simulink library "Model_DG_Grid_Forming_Converter"  (R2022b)
settings: Solver=VariableStepAuto  StartTime=0.0  StopTime=10.0  RelTol=1e-3
settings Model: Creator=winkens  LastModifiedBy=winkens
settings SolverCC: AlgebraicLoopSolver=TrustRegion
settings DebuggingCC: UnconnectedInputMsg=warning  UnconnectedOutputMsg=warning  UnconnectedLineMsg=warning  SFMachineParentedDataDiag=warning
settings ModelReferenceCC: EnableRefExpFcnMdlSchedulingChecks=on
settings RTWCC: DLArmComputeVersion=19.05

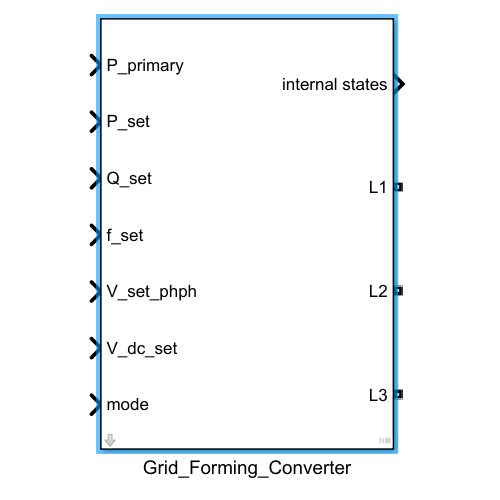
[thumbnail: Simulink's stored preview of the top-level diagram]
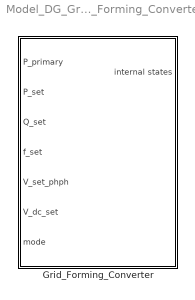
== system Model_DG_Grid_Forming_Converter ==
  Grid_Forming_Converter : Subsystem  mask{S_n=2e6, V_n_phph=690, f_n=50, send_messages=on, T_s_ctrl=1e-4, T_s_PWM_meas=1e-4, T_s_SPS=1e-4, datatype='double', swModeling=Average Model, f_sw=5e3, L_filter_conv_pu=[ 0.001 0.05097 ], C_filter_pu=[ 0.06875 0.04569 ], L_filter_grid_pu=[ 0.01 0.04 ], C_dc_pu=0.75, withTransformer=Grid coupling using transformer, V_n_grid_phph=20e3, RL_Trafo_Conv=[ 0.005 0.02 ], RL_Trafo_Grid=[ 0.005 0.02 ], Rm=500, Lm=500, meas_lowpass=on, meas_f_cutoff_lowpass=2500, meas_f_cutoff_posseq=20, prot_variant=VDE AR, v_dc_max=1.2, v_ac_max=1.4, t_ac_max=0.1, v_ac_maxmax=1.25, t_ac_maxmax=0.1, v_ac_min=0.8, t_ac_min=3, v_ac_minmin=0.45, t_ac_minmin=0.3, f_ac_max=51.5, t_f_ac_max=0.1, f_ac_maxmax=52.5, t_f_ac_maxmax=10, f_ac_min=47.5, t_f_ac_min=0.1, i_ac_max=1.3, outerCtrlStrategy=Droop, OuterCtrl_droop_kP=0.05, OuterCtrl_droop_kQ=0.1, OuterCtrl_droop_TQ=0.2, OuterCtrl_ZDroop_kf=0.05, OuterCtrl_ZDroop_kV=0.1, OuterCtrl_ZDroop_kR=0, OuterCtrl_ZDroop_kX=1, OuterCtrl_ZDroop_TV=0.2, OuterCtrl_VSM_H=0.1, OuterCtrl_VSM_Kd=40, OuterCtrl_VSM_K=20, OuterCtrl_VSM_kQ=0.1, OuterCtrl_VSM_TQ=0.2, OuterCtrl_Dual_Kp=0.01, OuterCtrl_Dual_Kd=1e-4, OuterCtrl_Dual_kQ=0.1, OuterCtrl_Dual_TQ=0.2, OuterCtrl_Lvirt=0, InnerCtrl_K_p_V_cap_controller=0.8, InnerCtrl_K_i_V_cap_controller=0.5, InnerCtrl_K_p_I_conv_controller=3.3, InnerCtrl_K_i_I_conv_controller=16.5, InnerCtrl_v_conv_max=1.3, InnerCtrl_i_conv_max=1, InnerCtrl_Cff_V_cap_ctrl=disabled, InnerCtrl_Cff_I_conv_ctrl=disabled, InnerCtrl_K_ff_I_grid=enabled, InnerCtrl_K_ff_V_cap=enabled, InnerCtrl_i_lim_type=dq coordinate system, InnerCtrl_active_damping=enabled, InnerCtrl_AD_R_virt_pu=0.2}
      mask prompts: S_n "Nominal Apparent Power [VA]"; V_n_phph "Nominal Converter Voltage (rms, phase-to-phase) [V]"; f_n "Nominal Frequency [Hz]"; send_messages "Send tDMSquared info messages"; T_s_ctrl "Controller sample time [s]"; T_s_PWM_meas "PWM and measurements sample time [s]"; T_s_SPS "Simscape SPS sample time [s]"; datatype "Signal data type"; swModeling "Model type:"; f_sw "Switching Frequency [Hz]:"; L_filter_conv_pu "Impedance of Converter-Side-Inductor [ R L ] (p.u.)"; C_filter_pu "Impedance of Filter Capacitor [ R C ] (p.u.)"; L_filter_grid_pu "Impedance of Grid-Side-Inductor* [ R L ] (p.u.)"; C_dc_pu "Capacitance of DC-Side-Capacitor [p.u.]"; V_n_grid_phph "Nominal Grid Voltage (rms, phase-to-phase) [V]"; RL_Trafo_Conv "Converter-Side Impedance [ R L ] (pu):"; RL_Trafo_Grid "Grid-Side Impedance [ R L ] (pu):"; Rm "Magnetization resistance Rm (pu):"; Lm "Magnetization inductance Lm (pu):"; meas_lowpass "Apply low pass filtering to measured signals"; meas_f_cutoff_lowpass "Cutoff-frequency of low pass filter applied to measurement signals [Hz]"; meas_f_cutoff_posseq "Cutoff-frequency of low pass filter for pos. sequence calculation [Hz]"; prot_variant "Protection Variant"; v_dc_max "Maximum DC-link voltage [% nom. value]"; v_ac_max "Maximum AC voltage [% nom. value]"; t_ac_max "Maximum AC voltage timing [s]"; v_ac_maxmax "Upper Maximum AC voltage [% nom. value]"; t_ac_maxmax "Upper Maximum AC voltage timing [s]"; v_ac_min "Upper Minimum AC voltage [% nom. value]"; t_ac_min "Upper Minimum AC voltage timing [s]"; v_ac_minmin "Lower Minimum AC voltage [% nom. value]"; t_ac_minmin "Lower Minimum AC voltage timing [s]"; f_ac_max "Maximum AC frequency[Hz]"; t_f_ac_max "Maximum AC frequency timing [s]"; f_ac_maxmax "Upper Maximum AC frequency [Hz]"; t_f_ac_maxmax "Upper Maximum AC frequency timing [s]"; f_ac_min "Minimum AC frequency [Hz]"; t_f_ac_min "Minimum AC frequency timing [s]"; i_ac_max "Maximum AC current [% nom. value]"; outerCtrlStrategy "Grid-Forming Control Strategy"; OuterCtrl_droop_kP "Droop constant kP (df[pu]/dP[pu])"; OuterCtrl_droop_kQ "Droop constant kQ (dV[pu]/dQ[pu])"; OuterCtrl_droop_TQ "PT1 time constant for QV-loop [s]"; OuterCtrl_ZDroop_kf "Droop constant kf (df/(dP+dQ))"; OuterCtrl_ZDroop_kV "Droop constant kV (dV/(dP+dQ))"; OuterCtrl_ZDroop_kR "R/Z-ratio"; OuterCtrl_ZDroop_kX "X/Z-ratio"; OuterCtrl_ZDroop_TV "PT1 time constant for voltage loop [s]"; OuterCtrl_VSM_H "Virtual inertia [s]"; OuterCtrl_VSM_Kd "Damping constant Kd [pu]"; OuterCtrl_VSM_K "Droop constant (dT/df) [pu]"; OuterCtrl_VSM_kQ "Droop constant kQ (dV/dQ)"; OuterCtrl_VSM_TQ "PT1 time constant QV-loop TQ [s]"; OuterCtrl_Dual_Kp "Proportional gain [pu]"; OuterCtrl_Dual_Kd "Derivative gain [pu]"; OuterCtrl_Dual_kQ "Droop constant kQ (dV/dQ)"; OuterCtrl_Dual_TQ "PT1 time constant QV-loop TQ [s]"; OuterCtrl_Lvirt "Virtual output inductance [pu]"; InnerCtrl_K_p_V_cap_controller "Proportional Gain (PI Voltage Controller)"; InnerCtrl_K_i_V_cap_controller "Integral Gain (PI Voltage Controller)"; InnerCtrl_K_p_I_conv_controller "Proportional Gain (PI Current Controller)"; InnerCtrl_K_i_I_conv_controller "Integral Gain (PI Current Controller)"; InnerCtrl_v_conv_max "Converter voltage maximum value (limit) [p.u.]"; InnerCtrl_i_conv_max "Converter current maximum value (limit) [p.u.]"; InnerCtrl_Cff_V_cap_ctrl "Command-feed-forward (Voltage Controller):"; InnerCtrl_Cff_I_conv_ctrl "Command-feed-forward (Current Controller):"; InnerCtrl_K_ff_I_grid "Current-feed-forward (Voltage Controller):"; InnerCtrl_K_ff_V_cap "Voltage-feed-forward (Current Controller):"; InnerCtrl_i_lim_type "Coordinate system of current setpoint limiter:"; InnerCtrl_active_damping "Active Damping"; InnerCtrl_AD_R_virt_pu "Virtual resistor (in series with converter-side inductance) [p.u.]"
      mask init:
      | % Initialize nominal grid voltage
      | if (withTransformer == 1)
      |     V_n_grid_phph = V_n_phph;
      | end
      mask TypeOptions swModeling: Ideal Switches | Average Model
      mask TypeOptions withTransformer: Direct grid coupling of converter | Grid coupling using transformer
      mask Callback withTransformer:
      | msk = Simulink.Mask.get(gcb);
      | p = msk.Parameters;
      | if strcmp(get_param(gcb, 'withTransformer'), 'Grid coupling using transformer')
      |     %with Transformer
      |     p(16).Visible = 'on';
      |     p(17).Visible = 'on';
      |     p(18).Visible = 'on';
      |     p(19).Visible = 'on';
      |     p(20).Visible = 'on';
      | else
      |     %without Transformer
      |     p(16).Visible = 'off';
      |     p(17).Visible = 'off';
      |     p(18).Visible = 'off';
      |     p(19).Visible = 'off';
      |     p(20).Visible = 'off';
      | end
      mask TypeOptions prot_variant: Hardware protection | tDMSquared warnings only | deactivated | VDE AR
      mask Callback prot_variant:
      | msk = Simulink.Mask.get(gcb);
      | if strcmp(get_param(gcb, 'prot_variant'), 'VDE AR')
      |     msk.getParameter('v_ac_max').Visible ='on';
      |     msk.getParameter('i_ac_max').Visible ='on';
      |     msk.getParameter('t_ac_max').Visible = 'on';
      |     msk.getParameter('v_ac_maxmax').Visible = 'on';
      |     msk.getParameter('t_ac_maxmax').Visible = 'on';
      |     msk.getParameter('v_ac_min').Visible = 'on';
      |     msk.getParameter('t_ac_min').Visible = 'on';
      |     msk.getParameter('v_ac_minmin').Visible = 'on';
      |     msk.getParameter('t_ac_minmin').Visible = 'on';
      |     msk.getParameter('f_ac_max').Visible = 'on';
      |     msk.getParameter('t_f_ac_max').Visible = 'on';
      |     msk.getParameter('f_ac_maxmax').Visible = 'on';
      |     msk.getParameter('t_f_ac_maxmax').Visible = 'on';
      |     msk.getParameter('f_ac_min').Visible = 'on';
      |     msk.getParameter('t_f_ac_min').Visible = 'on';
      | elseif strcmp(get_param(gcb, 'prot_variant'), 'deactivated')
      |     msk.getParameter('v_ac_max').Visible ='off';
      |     msk.getParameter('i_ac_max').Visible ='off';
      |     msk.getParameter('t_ac_max').Visible = 'off';
      |     msk.getParameter('v_ac_maxmax').Visible = 'off';
      |     msk.getParameter('t_ac_maxmax').Visible = 'off';
      |     msk.getParameter('v_ac_min').Visible = 'off';
      |     msk.getParameter('t_ac_min').Visible = 'off';
      |     msk.getParameter('v_ac_minmin').Visible = 'off';
      |     msk.getParameter('t_ac_minmin').Visible = 'off';
      |     msk.getParameter('f_ac_max').Visible = 'off';
      |     msk.getParameter('t_f_ac_max').Visible = 'off';
      |     msk.getParameter('f_ac_maxmax').Visible = 'off';
      |     msk.getParameter('t_f_ac_maxmax').Visible = 'off';
      |     msk.getParameter('f_ac_min').Visible = 'off';
      |     msk.getParameter('t_f_ac_min').Visible = 'off';
      | else
      |     msk.getParameter('v_ac_max').Visible ='on';
      |     msk.getParameter('i_ac_max').Visible ='on';
      |     msk.getParameter('t_ac_max').Visible = 'off';
      |     msk.getParameter('v_ac_maxmax').Visible = 'off';
      |     msk.getParameter('t_ac_maxmax').Visible = 'off';
      |     msk.getParameter('v_ac_min').Visible = 'off';
      |     msk.getParameter('t_ac_min').Visible = 'off';
      |     msk.getParameter('v_ac_minmin').Visible = 'off';
      |     msk.getParameter('t_ac_minmin').Visible = 'off';
      |     msk.getParameter('f_ac_max').Visible = 'off';
      |     msk.getParameter('t_f_ac_max').Visible = 'off';
      |     msk.getParameter('f_ac_maxmax').Visible = 'off';
      |     msk.getParameter('t_f_ac_maxmax').Visible = 'off';
      |     msk.getParameter('f_ac_min').Visible = 'off';
      |     msk.getParameter('t_f_ac_min').Visible = 'off';
      | end
      mask TypeOptions outerCtrlStrategy: Droop | Impedance-dependent droop | Virtual Synchronous Machine (VSM) | Dual-Port Grid-Forming Control
      mask TypeOptions InnerCtrl_Cff_V_cap_ctrl: disabled | enabled
      mask TypeOptions InnerCtrl_Cff_I_conv_ctrl: disabled | enabled
      mask TypeOptions InnerCtrl_K_ff_I_grid: disabled | enabled
      mask TypeOptions InnerCtrl_K_ff_V_cap: disabled | enabled
      mask TypeOptions InnerCtrl_i_lim_type: dq coordinate system | abc coordinate system
      mask TypeOptions InnerCtrl_active_damping: disabled | enabled
      mask DialogControl DescGroupVar Prompt: Grid-Forming Converter
      mask DialogControl DescTextVar Prompt: Three-phase converter model based on different grid-forming control strategies. Power electronics can either be modeled as switches or as average model.
      mask DialogControl Container19 Prompt: General
      mask DialogControl Container42 Prompt: Sample Times and Data Types
      mask DialogControl Container30 Prompt: Electrical Part
      mask DialogControl pwmGenParam Prompt: Modeling of Switches
      mask DialogControl Container36 Prompt: Filter and DC components
      mask DialogControl Control4_copy Prompt: The filter parameters are defined in a per-unit-system based on the nominal power, the nominal frequency and the nominal converter-side voltage defined in tab General.
      mask DialogControl Control5 Prompt: *Only if no transformer is used.
      mask DialogControl TransformerParams Prompt: Transformer parameters
      mask DialogControl Control4 Prompt: Transformer parameters are defined in a per-unit-system based on the nominal power, the nominal frequency and the nominal voltages defined here and in tab General. The reference voltage for the impedance values depends on the respective nominal voltage level. However, magnetization resistance and inductance are based on the generator-side nominal voltage.
      mask DialogControl Container26 Prompt: Measurements
      mask DialogControl Control6 Prompt: These parameters are related to the processing of the measurement signals.
      mask DialogControl Container41 Prompt: Protection Parameters
      mask DialogControl Container31 Prompt: Grid-Forming Control
      mask DialogControl Container13 Prompt: Droop
      mask DialogControl Container21 Prompt: Z-dependent droop
      mask DialogControl Container22 Prompt: VSM
      mask DialogControl Container50 Prompt: Dual-Port
      mask DialogControl Container49 Prompt: Virtual Inductance
      mask DialogControl Container32 Prompt: Inner Control
      mask DialogControl Container34 Prompt: Cascaded PI Controller
      mask DialogControl Container10 Prompt: Basic
      mask DialogControl Container11 Prompt: Advanced
      mask DialogControl Container39 Prompt: Active Damping

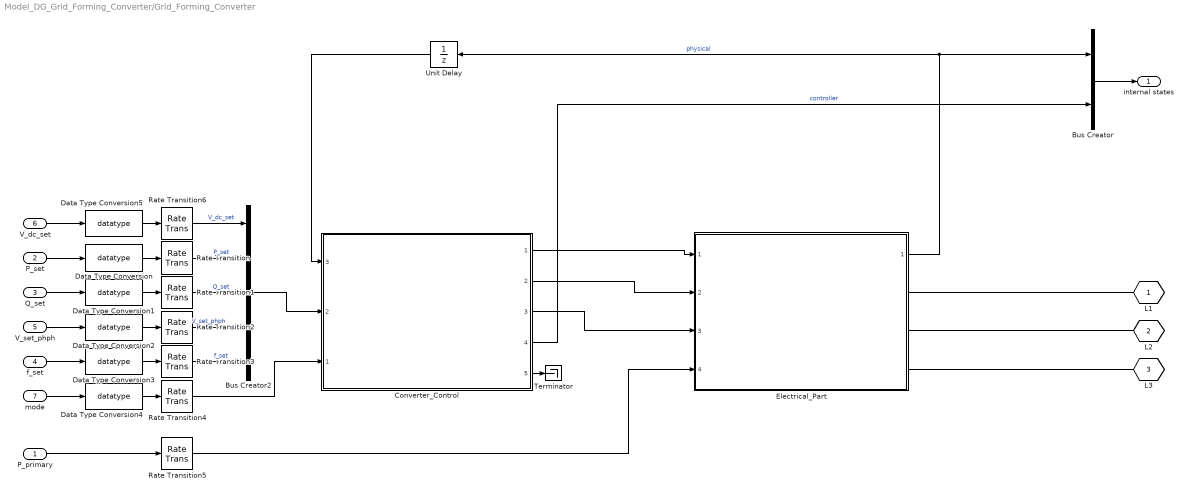
== system Model_DG_Grid_Forming_Converter/Grid_Forming_Converter ==
  P_primary : Inport  PortDimensions=1
  P_set : Inport  Port=2  PortDimensions=1
  Q_set : Inport  Port=3  PortDimensions=1
  f_set : Inport  Port=4  PortDimensions=1
  V_set_phph : Inport  Port=5  PortDimensions=1
  V_dc_set : Inport  Port=6  PortDimensions=1
  mode : Inport  Port=7  PortDimensions=1
  Bus Creator : BusCreator  Inputs=2
  Bus Creator2 : BusCreator  Inputs=5
  Converter_Control : Subsystem  ReferencedSubsystem=Subsys_GFormConv_Control  S_n=S_n  f_n=f_n  V_n_phph=V_n_phph  V_n_grid_phph=V_n_grid_phph  V_n_dc=2*V_n_phph  RL_filter_conv_pu=L_filter_conv_pu  RC_filter_pu=C_filter_pu  outputSignal=2 - swModeling  f_sw=f_sw  sendInfoMessages=send_messages  T_s_ctrl=T_s_ctrl  T_s_PWM_meas=T_s_PWM_meas  datatype=datatype  meas_signals=0  meas_noise_filter=meas_lowpass  f_cutoff_meas=meas_f_cutoff_lowpass  f_cutoff_posseq=meas_f_cutoff_posseq  prot_variant=prot_variant  v_dc_max=v_dc_max  v_ac_max=v_ac_max  t_ac_max=t_ac_max  v_ac_maxmax=v_ac_maxmax  t_ac_maxmax=t_ac_maxmax  v_ac_min=v_ac_min  t_ac_min=t_ac_min  v_ac_minmin=v_ac_minmin  t_ac_minmin=t_ac_minmin  f_ac_max=f_ac_max  t_f_ac_max=t_f_ac_max  f_ac_maxmax=f_ac_maxmax  t_f_ac_maxmax=t_f_ac_maxmax  f_ac_min=f_ac_min  t_f_ac_min=t_f_ac_min  i_ac_max=i_ac_max  OuterCtrlStrategy=outerCtrlStrategy - 1  OuterCtrl_Droop_kP=OuterCtrl_droop_kP  OuterCtrl_Droop_kQ=OuterCtrl_droop_kQ  OuterCtrl_Droop_TQ=OuterCtrl_droop_TQ  OuterCtrl_ZDroop_kf=OuterCtrl_ZDroop_kf  OuterCtrl_ZDroop_kV=OuterCtrl_ZDroop_kV  OuterCtrl_ZDroop_kR=OuterCtrl_ZDroop_kR  OuterCtrl_ZDroop_kX=OuterCtrl_ZDroop_kX  OuterCtrl_ZDroop_TV=OuterCtrl_ZDroop_TV  OuterCtrl_Dual_Kp=OuterCtrl_Dual_Kp  OuterCtrl_Dual_Kd=OuterCtrl_Dual_Kd  OuterCtrl_Dual_kQ=OuterCtrl_Dual_kQ  OuterCtrl_Dual_TQ=OuterCtrl_Dual_TQ  OuterCtrl_VSM_H=OuterCtrl_VSM_H  OuterCtrl_VSM_Kd=OuterCtrl_VSM_Kd  OuterCtrl_VSM_K=OuterCtrl_VSM_K  OuterCtrl_VSM_kQ=OuterCtrl_VSM_kQ  OuterCtrl_VSM_TQ=OuterCtrl_VSM_TQ  L_virt=OuterCtrl_Lvirt  active_damping=InnerCtrl_active_damping - 1  R_virt_pu=InnerCtrl_AD_R_virt_pu  InnerCtrl_K_p_v_cap=InnerCtrl_K_p_V_cap_controller  InnerCtrl_K_i_v_cap=InnerCtrl_K_i_V_cap_controller  InnerCtrl_K_p_i_conv=InnerCtrl_K_p_I_conv_controller  InnerCtrl_K_i_i_conv=InnerCtrl_K_i_I_conv_controller  InnerCtrl_C_ff_v_cap_ctrl=InnerCtrl_Cff_V_cap_ctrl - 1  InnerCtrl_C_ff_i_conv_ctrl=InnerCtrl_Cff_I_conv_ctrl - 1  InnerCtrl_K_ff_i=InnerCtrl_K_ff_I_grid - 1  InnerCtrl_K_ff_v=InnerCtrl_K_ff_V_cap - 1  InnerCtrl_i_conv_max=InnerCtrl_i_conv_max  InnerCtrl_v_conv_max=InnerCtrl_v_conv_max  InnerCtrl_i_lim_type=InnerCtrl_i_lim_type - 1
      settings: PortSchema="{\"entries\":[{\"content\":{\"sides\":[{\"content\":{\"connectorIds\":[\"In3\",\"In2\",\"In1\"]},\"type\":\"ConnectorPlacement.EquallySpacedRectSide\",\"uuid\":\"ae610b2f-473b-4f6d-8877-a2052ccbf331\"},{\"content\":{\"connectorIds\":[\"Out1\",\"Out2\",\"Out3\",\"Out4\",\"Out5\"],\"side\":\"RIGHT\"},\"type\":\"ConnectorPlacement.EquallySpacedRectSide\",\"uuid\":\"ca06f4e3-2aff-495b-9872-f5836059196f\"},{\"content\":{\"connectorIds\":[],\"side\":\"TOP\"},\"type\":\"ConnectorPlacement.EquallySpacedRectSide\",\"uuid\":\"0b816637-2513-44ba-956e-b9da96b1cff8\"},{\"content\":{\"connectorIds\":[],\"side\":\"HIDDEN\"},\"type\":\"ConnectorPlacement.EquallySpacedRectSide\",\"uuid\":\"342141a1-ab21-488b-8110-74f7bef3c4d4\"}]},\"type\":\"ConnectorPlacement.EquallySpacedConnector\",\"uuid\":\"f643e82e-2ffb-4562-aabe-68d7cb8bf533\"}],\"packageUris\":[\"http://schema.mathworks.com/mf0/Connector/R2020b\"],\"version\":\"1.0\"}"
  Data Type Conversion{,1..5} (6 alike) : DataTypeConversion  OutDataTypeStr=datatype  SaturateOnIntegerOverflow=off  RndMeth=Floor
  Electrical_Part : Subsystem  ReferencedSubsystem=Subsys_Conv_Electrical_Part_SPS  S_n=S_n  f_n=f_n  V_n_phph=V_n_phph  V_n_grid_phph=V_n_grid_phph  T_s_ctrl=T_s_ctrl  T_s_meas=T_s_PWM_meas  T_s_SPS=T_s_SPS  datatype=datatype  L_filter_conv_pu=L_filter_conv_pu  C_filter_pu=C_filter_pu  L_filter_grid_pu=L_filter_grid_pu  withTransformer=withTransformer - 1  RL_Trafo_Conv=RL_Trafo_Conv  RL_Trafo_Grid=RL_Trafo_Grid  Rm=Rm  Lm=Lm  inverterModel=swModeling - 1  R_snubber_pu=5e6  R_on_pu=1e-3  energySourceModel=1  C_dc_pu=C_dc_pu  K_p_DC=1.2  K_i_DC=2.4
  Rate Transition{,1..6} (7 alike) : RateTransition  OutPortSampleTime=T_s_ctrl
  Terminator : Terminator
  Unit Delay : UnitDelay  SampleTime=-1  HasFrameUpgradeWarning=on
  L1 : PMIOPort  Tag=PMCPort  Side=Right
  L2 : PMIOPort  Tag=PMCPort  Port=2  Side=Right
  L3 : PMIOPort  Tag=PMCPort  Port=3  Side=Right
  internal states : Outport
  wires:
  P_set/1 -> Data Type Conversion/1
  Q_set/1 -> Data Type Conversion1/1
  f_set/1 -> Data Type Conversion3/1
  V_set_phph/1 -> Data Type Conversion2/1
  Bus Creator2/1 -> Converter_Control/2
  Converter_Control/4 -> Bus Creator/2  "controller"
  Bus Creator/1 -> internal states/1
  mode/1 -> Data Type Conversion4/1
  Converter_Control/3 -> Electrical_Part/3
  Electrical_Part/1 -> Bus Creator/1, Unit Delay/1  "physical"
  Converter_Control/1 -> Electrical_Part/1
  Converter_Control/2 -> Electrical_Part/2
  Unit Delay/1 -> Converter_Control/3
  Converter_Control/5 -> Terminator/1
  Data Type Conversion/1 -> Rate Transition/1
  Data Type Conversion1/1 -> Rate Transition1/1
  Data Type Conversion2/1 -> Rate Transition2/1
  Data Type Conversion3/1 -> Rate Transition3/1
  Data Type Conversion4/1 -> Rate Transition4/1
  P_primary/1 -> Rate Transition5/1
  Rate Transition/1 -> Bus Creator2/2  "P_set"
  Rate Transition1/1 -> Bus Creator2/3  "Q_set"
  Rate Transition2/1 -> Bus Creator2/4  "V_set_phph"
  Rate Transition3/1 -> Bus Creator2/5  "f_set"
  Rate Transition4/1 -> Converter_Control/1
  Rate Transition5/1 -> Electrical_Part/4
  V_dc_set/1 -> Data Type Conversion5/1
  Data Type Conversion5/1 -> Rate Transition6/1
  Rate Transition6/1 -> Bus Creator2/1  "V_dc_set"
  connections:
  Electrical_Part/RConn1 -- L1/RConn1
  Electrical_Part/RConn2 -- L2/RConn1
  Electrical_Part/RConn3 -- L3/RConn1
